simulink model "can_encoder"  (R2023b)
settings: Solver=FixedStepDiscrete  StartTime=0.0  StopTime=0.1  FixedStep=Ts_can_encoder  RelTol=1e-3  EnableMultiTasking=on
undefined symbols (not defined in the file): CAN_ANGLE_DEG2ICUB, CAN_ID_AMC, CAN_VOLT_REF_GAIN, CAN_VOLT_REF_SHIFT
settings Model: DataDictionary=EmbeddedBoardDD.sldd  Creator=upattacini  LastModifiedBy=upattacini
settings SolverCC: AllowMultiTaskInputOutput=on  AutoInsertRateTranBlk=on  InsertRTBMode=Never (minimum delay)
settings DataIOCC: SaveOutput=off  SignalLogging=off  DSMLogging=off  SaveTime=off  ReturnWorkspaceOutputs=off
settings OptimizationCC: DefaultParameterBehavior=Inlined  DefaultUnderspecifiedDataType=single  StrengthReduction=on  PassReuseOutputArgsAs=Individual arguments  ZeroExternalMemoryAtStartup=off  ZeroInternalMemoryAtStartup=off  OptimizeBlockOrder=speed  OptimizationPriority=Speed  OptimizationCustomize=off  MultiThreadedLoops=on  EfficientTunableParamExpr=on
settings DebuggingCC: ParameterPrecisionLossMsg=none  UnconnectedInputMsg=warning  UnconnectedOutputMsg=warning  UnconnectedLineMsg=warning
settings HardwareCC: ProdBitPerPointer=32  ProdBitPerSizeT=32  ProdBitPerPtrDiffT=32  ProdLargestAtomicInteger=Long  ProdLargestAtomicFloat=Double  ProdWordSize=32  ProdHWDeviceType=ARM Compatible->ARM Cortex-M
settings ModelReferenceCC: UpdateModelReferenceTargets=Force  EnableRefExpFcnMdlSchedulingChecks=on  ModelReferenceNumInstancesAllowed=Single
settings SFSimCC: MATLABDynamicMemAlloc=off
settings RTWCC: Description=Embedded Coder  SystemTargetFile=ert.tlc  GenCodeOnly=on  PackageGeneratedCodeAndArtifacts=on  PackageName=can_encoder  TemplateMakefile=ert_default_tmf  GenerateReport=on  LaunchReport=on  TargetLang=C++  GenerateCodeReplacementReport=on  DLArmComputeVersion=19.05
settings CodeAppCC: ForceParamTrailComments=on  IgnoreCustomStorageClasses=off  MaxIdLength=60  OperatorAnnotations=on  SimulinkDataObjDesc=on  SFDataObjDesc=on  InsertBlockDesc=on
settings ERTTargetCC: TargetLangStandard=C++03 (ISO)  CodeReplacementLibrary=ARM Cortex-M,iCubTech  GenerateSampleERTMain=on  SupportVariableSizeSignals=on  InlinedParameterPlacement=NonHierarchical  RootIOFormat=Structure reference  ERTCustomFileTemplate=example_file_process.tlc

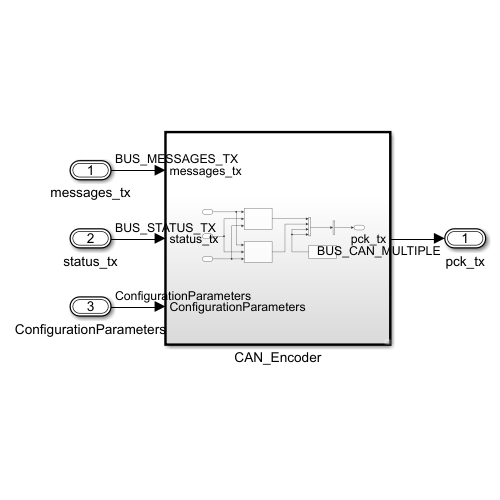
[thumbnail: Simulink's stored preview of the top-level diagram]
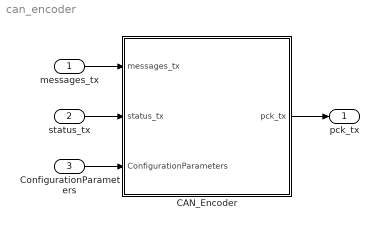
== system can_encoder ==
  messages_tx : Inport  OutDataTypeStr=Bus: BUS_MESSAGES_TX  BusOutputAsStruct=on
  status_tx : Inport  Port=2  OutDataTypeStr=Bus: BUS_STATUS_TX  BusOutputAsStruct=on
  ConfigurationParameters : Inport  Port=3  OutDataTypeStr=Bus: ConfigurationParameters  BusOutputAsStruct=on
  CAN_Encoder : Subsystem  TreatAsAtomicUnit=on
  pck_tx : Outport  OutDataTypeStr=Bus: BUS_CAN_MULTIPLE  BusOutputAsStruct=on
  wires:
  messages_tx/1 -> CAN_Encoder/1(messages_tx)
  status_tx/1 -> CAN_Encoder/2(status_tx)
  CAN_Encoder/1(pck_tx) -> pck_tx/1
  ConfigurationParameters/1 -> CAN_Encoder/3(ConfigurationParameters)

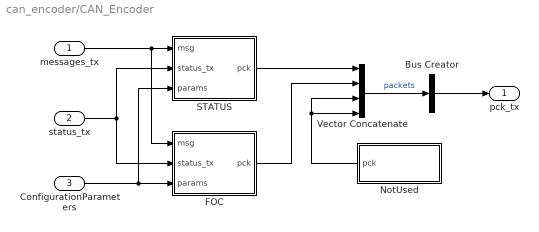
== system can_encoder/CAN_Encoder ==
  messages_tx : Inport  OutDataTypeStr=Bus: BUS_MESSAGES_TX
  status_tx : Inport  Port=2  OutDataTypeStr=Bus: BUS_STATUS_TX
  ConfigurationParameters : Inport  Port=3  OutDataTypeStr=Bus: ConfigurationParameters
  Bus Creator : BusCreator  Inputs=1  OutDataTypeStr=Bus: BUS_CAN_MULTIPLE  NonVirtualBus=on
      settings: InheritFromInputs=off
  FOC : Subsystem
  NotUsed : Subsystem
  STATUS : Subsystem
  Vector Concatenate : Concatenate  NumInputs=CAN_MAX_NUM_PACKETS
  pck_tx : Outport
  wires:
  Bus Creator/1 -> pck_tx/1
  Vector Concatenate/1 -> Bus Creator/1  "packets"
  NotUsed/1(pck) -> Vector Concatenate/4, Vector Concatenate/3
  FOC/1(pck) -> Vector Concatenate/2
  STATUS/1(pck) -> Vector Concatenate/1
  messages_tx/1 -> STATUS/1(msg), FOC/1(msg)
  status_tx/1 -> FOC/2(status_tx), STATUS/2(status_tx)
  ConfigurationParameters/1 -> FOC/3(params), STATUS/3(params)

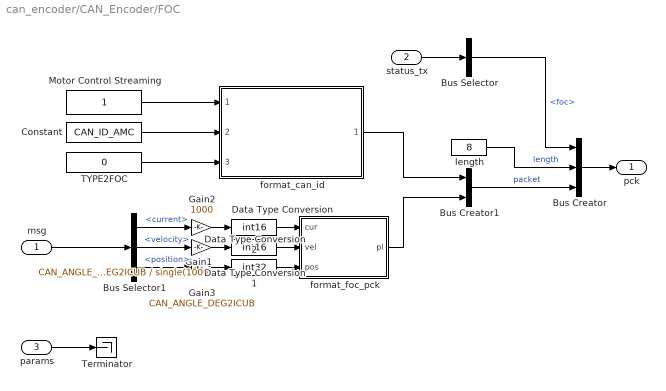
== system can_encoder/CAN_Encoder/FOC ==
  msg : Inport
  status_tx : Inport  Port=2
  params : Inport  Port=3
  Bus Creator : BusCreator  Inputs=3  OutDataTypeStr=Bus: BUS_CAN  NonVirtualBus=on
      settings: InheritFromInputs=off
  Bus Creator1 : BusCreator  Inputs=2  OutDataTypeStr=Bus: BUS_CAN_PACKET  NonVirtualBus=on
      settings: InheritFromInputs=off
  Bus Selector : BusSelector  OutputSignals=foc
  Bus Selector1 : BusSelector  OutputSignals=foc.current,foc.velocity,foc.position
  Constant : Constant  Value=CAN_ID_AMC
  Data Type Conversion : DataTypeConversion  OutDataTypeStr=int16  RndMeth=Simplest
  Data Type Conversion1 : DataTypeConversion  OutDataTypeStr=int16  RndMeth=Simplest
  Data Type Conversion2 : DataTypeConversion  OutDataTypeStr=int32  RndMeth=Simplest
  Gain1 : Gain  Gain=CAN_ANGLE_DEG2ICUB / single(1000)
  Gain2 : Gain  Gain=1000
  Gain3 : Gain  Gain=CAN_ANGLE_DEG2ICUB
  Motor Control Streaming : Constant  OutDataTypeStr=uint8
  TYPE2FOC : Constant  Value=0  OutDataTypeStr=uint8
  Terminator : Terminator
  format_can_id : Subsystem  ReferencedSubsystem=format_can_id
  format_foc_pck : MATLAB Function  TreatAsAtomicUnit=on
  length : Constant  Value=8  OutDataTypeStr=uint8
  pck : Outport
  wires:
  Bus Selector1/3 -> Gain3/1  "<position>"
  format_foc_pck/1(pl) -> Bus Creator1/2
  Bus Selector1/1 -> Gain2/1  "<current>"
  Bus Selector1/2 -> Gain1/1  "<velocity>"
  Gain2/1 -> Data Type Conversion/1
  msg/1 -> Bus Selector1/1
  Motor Control Streaming/1 -> format_can_id/1
  Constant/1 -> format_can_id/2
  TYPE2FOC/1 -> format_can_id/3
  format_can_id/1 -> Bus Creator1/1
  Bus Creator1/1 -> Bus Creator/3  "packet"
  Bus Creator/1 -> pck/1
  length/1 -> Bus Creator/2  "length"
  status_tx/1 -> Bus Selector/1
  Bus Selector/1 -> Bus Creator/1  "<foc>"
  Data Type Conversion/1 -> format_foc_pck/1(cur)
  Data Type Conversion1/1 -> format_foc_pck/2(vel)
  Data Type Conversion2/1 -> format_foc_pck/3(pos)
  Gain1/1 -> Data Type Conversion1/1
  Gain3/1 -> Data Type Conversion2/1
  params/1 -> Terminator/1

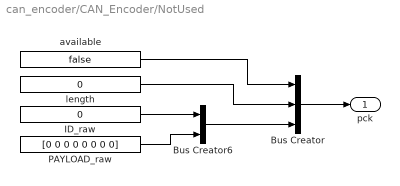
== system can_encoder/CAN_Encoder/NotUsed ==
  Bus Creator : BusCreator  Inputs=3  OutDataTypeStr=Bus: BUS_CAN  NonVirtualBus=on
      settings: InheritFromInputs=off
  Bus Creator6 : BusCreator  Inputs=2  OutDataTypeStr=Bus: BUS_CAN_PACKET  NonVirtualBus=on
      settings: InheritFromInputs=off
  ID_raw : Constant  Value=0  OutDataTypeStr=uint16
  PAYLOAD_raw : Constant  Value=[0 0 0 0 0 0 0 0]  OutDataTypeStr=uint8
  available : Constant  Value=false  OutDataTypeStr=boolean
  length : Constant  Value=0  OutDataTypeStr=uint8
  pck : Outport
  wires:
  ID_raw/1 -> Bus Creator6/1
  PAYLOAD_raw/1 -> Bus Creator6/2
  Bus Creator6/1 -> Bus Creator/3
  Bus Creator/1 -> pck/1
  available/1 -> Bus Creator/1
  length/1 -> Bus Creator/2

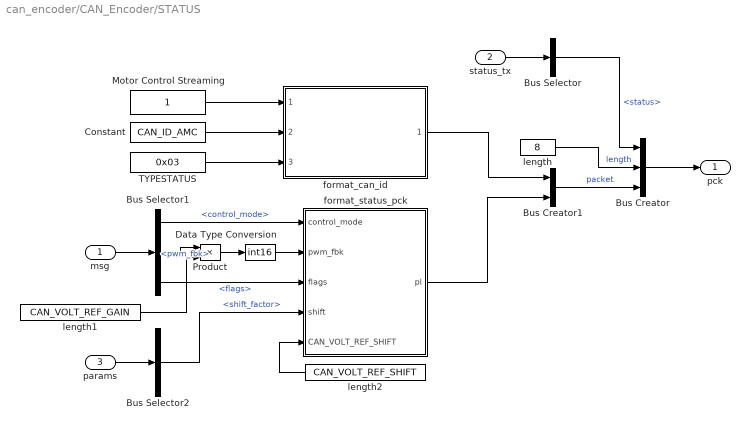
== system can_encoder/CAN_Encoder/STATUS ==
  msg : Inport
  status_tx : Inport  Port=2
  params : Inport  Port=3
  Bus Creator : BusCreator  Inputs=3  OutDataTypeStr=Bus: BUS_CAN  NonVirtualBus=on
      settings: InheritFromInputs=off
  Bus Creator1 : BusCreator  Inputs=2  OutDataTypeStr=Bus: BUS_CAN_PACKET  NonVirtualBus=on
      settings: InheritFromInputs=off
  Bus Selector : BusSelector  OutputSignals=status
  Bus Selector1 : BusSelector  OutputSignals=status.control_mode,status.pwm_fbk,status.flags
  Bus Selector2 : BusSelector  OutputSignals=CurLoopPID.shift_factor
  Constant : Constant  Value=CAN_ID_AMC
  Data Type Conversion : DataTypeConversion  OutDataTypeStr=int16  RndMeth=Simplest
  Motor Control Streaming : Constant  OutDataTypeStr=uint8
  Product : Product
  TYPESTATUS : Constant  Value=0x03  OutDataTypeStr=uint8
  format_can_id : Subsystem  ReferencedSubsystem=format_can_id
  format_status_pck : MATLAB Function  TreatAsAtomicUnit=on
  length : Constant  Value=8  OutDataTypeStr=uint8
  length1 : Constant  Value=CAN_VOLT_REF_GAIN  OutDataTypeStr=single
  length2 : Constant  Value=CAN_VOLT_REF_SHIFT  OutDataTypeStr=uint8
  pck : Outport
  wires:
  msg/1 -> Bus Selector1/1
  Constant/1 -> format_can_id/2
  Motor Control Streaming/1 -> format_can_id/1
  format_can_id/1 -> Bus Creator1/1
  TYPESTATUS/1 -> format_can_id/3
  format_status_pck/1(pl) -> Bus Creator1/2
  Bus Selector1/1 -> format_status_pck/1(control_mode)  "<control_mode>"
  Data Type Conversion/1 -> format_status_pck/2(pwm_fbk)
  Bus Selector1/3 -> format_status_pck/3(flags)  "<flags>"
  Bus Selector/1 -> Bus Creator/1  "<status>"
  status_tx/1 -> Bus Selector/1
  Bus Creator1/1 -> Bus Creator/3  "packet"
  length/1 -> Bus Creator/2  "length"
  Bus Creator/1 -> pck/1
  params/1 -> Bus Selector2/1
  Bus Selector2/1 -> format_status_pck/4(shift)  "<shift_factor>"
  length2/1 -> format_status_pck/5(CAN_VOLT_REF_SHIFT)
  Bus Selector1/2 -> Product/1  "<pwm_fbk>"
  Product/1 -> Data Type Conversion/1
  length1/1 -> Product/2

== matlab function can_encoder/CAN_Encoder/FOC/format_foc_pck ==
  data: cur input; pl output; vel input; pos input
function pl = format_foc_pck(cur, vel, pos)

pl = uint8((zeros(8, 1)));

tmp = typecast(cur, 'uint8');
pl(1) = tmp(1);
pl(2) = tmp(2);

tmp = typecast(vel, 'uint8');
pl(3) = tmp(1);
pl(4) = tmp(2);

tmp = typecast(pos, 'uint8');
pl(5) = tmp(1);
pl(6) = tmp(2);
pl(7) = tmp(3);
pl(8) = tmp(4);

== matlab function can_encoder/CAN_Encoder/STATUS/format_status_pck ==
  data: control_mode input; pl output; pwm_fbk input; flags input; shift input; CAN_VOLT_REF_SHIFT input
function pl = format_status_pck(control_mode, pwm_fbk, flags, shift, CAN_VOLT_REF_SHIFT)

pl = uint8((zeros(8, 1)));

pl(1) = uint8(control_mode);

pl(2) = uint8(0);

tmp1 = bitshift(pwm_fbk, CAN_VOLT_REF_SHIFT - shift);
tmp2 = typecast(tmp1, 'uint8');
pl(3) = tmp2(1);
pl(4) = tmp2(2);

% See https://github.com/robotology/icub-firmware/blob/devel/emBODY/eBcode/arch-arm/board/amc2c/bsp/motorhal/motorhal_faults.h
pl(5) = bitset(pl(5), 1, flags.ExternalFaultAsserted);
pl(5) = bitset(pl(5), 4, flags.OverCurrentFailure);
pl(6) = uint8(0);
pl(7) = uint8(0);
pl(8) = uint8(0);
